simulink model "furuta_block_model_pi"  (R2026b)
settings: Solver=ode14x  StopTime=5  FixedStep=driveElectrical.sampleTime
model workspace (MAT data in the model file):
  controlPeriod = 0.01
  driveElectrical : object (value not decoded)
  furutaPPOAgent : rl.agent.rlPPOAgent (value not decoded)
  furutaSACAgent : rl.agent.rlSACAgent (value not decoded)
  furutaToolboxMpc : object (value not decoded)
  initialState = [0; 0.174532925199; 0; 0]
  integrationStep = 0.002
  lqrGain = [-0.560244322113 -7.30813603654 -0.304541725168 -0.68699829167]
  maxTorque = 0.03
  piReplayEnabled = 0
  piReplayState = [0  0  0  0  0; 5  0  0  0  0]
  pidGains = [7.30813603654 0.68699829167 0.560244322113 0.304541725168 0.01]
  plantCoefficients = [0.00019818 0.00016078 0.00016134 0.00013805 0.016934 0.0001 1e-05 0]
  rlRewardLevel = 2
  rmd : object (value not decoded)
  rmdCommandDelaySamples = 0
  scenarioStimulus = [0 0.0075 0.0175 0.0275 0.0375 0.0475 0.0575 0.0675 0.0775 0.0875 0.0975 0.1075 ... (2004 elements, 501x4)]
  usePolicyCallback = 0
  useRmd = 1
values from neighbouring files (symbols this model uses):
  C = [B A*B A^2*B A^3*B]    [build_furuta_rmd.m]
  N = 20    [build_furuta_rl.m]    (also in design_classical.m)
  s = load(matFile,'ds')    [analyze_pi_current_run.m]    (also in analyze_pi_speed_run.m; build_furuta_rl.m = sin(x(2));"; build_furuta_simulink.m = s(1); design_classical.m = furuta_scenarios)
  source = [step '/1']    [add_furuta_plant_blocks.m]    (also in build_furuta_pi.m = get_param(line,'SrcPortHandle'); build_furuta_pi_hardware.m = 'Drive interlocks/3'; compare_furuta_actuators.m = get_param([harness '/Requested torque'],'PortHandles'))
  Z = expm([A B; zeros(1,5)]*p.Ts)    [furuta_linearize.m]
symbols that are objects in the model workspace (value not decoded): driveElectrical, rmd
undefined symbols (not defined in the file or in its folder): lmpcF, lmpcH, poleGain, sgn, X, Y
libraries: sm_lib x36, nesl_utility x8, fl_lib x7, rllib x2, mpclib x1, slpidlib x1, ee_lib x1
(part 4 of 4)

== matlab function furuta_block_model_pi/03 Controllers/SAC/RL observation reward termination ==
  data: x input; obs output; lastAction input; level input; mode input; reward output; done output
function [obs,reward,done] = observe(x,lastAction,level,mode)
% 상태는 현재 샘플, 보상에 쓰는 행동은 이전 샘플이다.
stateVector = x(:);
active = mode == 4;
obs = zeros(5,1);
reward = 0;
done = false;
if ~active
    return
end
persistent startedUpright
if isempty(startedUpright)
    startedUpright = abs(atan2(sin(stateVector(2)),cos(stateVector(2))))<pi/9;
end
angle = abs(atan2(sin(stateVector(2)),cos(stateVector(2))));
if any(~isfinite(stateVector)) || abs(stateVector(1))>2*pi || max(abs(stateVector(3:4)))>30 || (startedUpright && angle>pi/4)
    done = true;
    reward = -50;
    return
end
c = cos(x(2)); s = sin(x(2));
obs = [c;s;x(1);x(3);x(4)];
reward = c-0.01*lastAction^2;
if level == 2
    reward = reward-.001*x(4)^2-.00002*x(3)^2+double(abs(atan2(s,c))<.35);
end
done = mode == 4 && abs(x(1))>2*pi;
if done
    reward = -50;
end
end

== matlab function furuta_block_model_pi/03 Controllers/LMPC (sim)/LMPC bounded QP ==
  data: x input; u output; mode input; H input; F input
function u = move(x,mode,H,F)
% 이전 해를 한 단계 이동해 재사용하고 모든 좌표를 [-1,1]로 제한한다.
persistent previous
if isempty(previous)
    previous = zeros(20,1);
end
u = 0;
if mode ~= 6
    previous(:) = 0;
    return
end
z = x(:);
z(2) = atan2(sin(z(2)),cos(z(2)));
f = F*z;
U = [previous(2:end); previous(end)];
gradient = H*U+f;
for it = 1:100
    change = 0;
    for j = 1:20
        next = min(1,max(-1,U(j)-gradient(j)/H(j,j)));
        step = next-U(j);
        U(j) = next;
        gradient = gradient+H(:,j)*step;
        change = max(change,abs(step));
    end
    if change<1e-7
        break
    end
end
previous = U;
u = U(1);
end

== matlab function furuta_block_model_pi/04 Actuator/RMD X6 P20 60 E/01 RMD Driver/Current PI and duty ==
  data: reference input; duty output; current input; emf input; p input; v output
function [duty,v] = regulate(reference,current,emf,p)
% 3상 등가 q축 전압 제한으로 정규화한 평균 브리지 지령.
persistent integral
if isempty(integral)
    integral = 0;
end
err = reference-current;
raw = emf+p(1)*err+integral;
vmax = p(4)/sqrt(3);
v = max(-vmax,min(vmax,raw));
if abs(raw)<=vmax || sign(raw)~=sign(err)
    integral = integral+p(2)*p(3)*err;
end
duty = .5+.5*v/p(4);
end

== matlab function furuta_block_model_pi/03 Controllers/PPO/RL observation reward termination ==
  data: x input; obs output; lastAction input; level input; mode input; reward output; done output
function [obs,reward,done] = observe(x,lastAction,level,mode)
% 상태는 현재 샘플, 보상에 쓰는 행동은 이전 샘플이다.
stateVector = mode(:);
active = x == 3;
obs = zeros(5,1);
reward = 0;
done = false;
if ~active
    return
end
persistent startedUpright
if isempty(startedUpright)
    startedUpright = abs(atan2(sin(stateVector(2)),cos(stateVector(2))))<pi/9;
end
angle = abs(atan2(sin(stateVector(2)),cos(stateVector(2))));
if any(~isfinite(stateVector)) || abs(stateVector(1))>2*pi || max(abs(stateVector(3:4)))>30 || (startedUpright && angle>pi/4)
    done = true;
    reward = -50;
    return
end
c = cos(mode(2)); s = sin(mode(2));
obs = [c;s;mode(1);mode(3);mode(4)];
reward = c-0.01*lastAction^2;
if level == 2
    reward = reward-.001*mode(4)^2-.00002*mode(3)^2+double(abs(atan2(s,c))<.35);
end
done = x == 3 && abs(mode(1))>2*pi;
if done
    reward = -50;
end
end
